simulink library "sm_pump_triplex_lib"  (R2025a)
settings: Solver=VariableStepAuto  StartTime=0.0  StopTime=10.0  RelTol=1e-3
undefined symbols (not defined in the file): cyl_stroke_P, seal_leak_vis_clr_P, seal_leak_vis_len_P, seal_leak_vis_rad_P, TRP_Par, X, Y, Z
libraries: sm_lib x30, fl_lib x10, SimscapeFluids_lib x4, nesl_utility x4
(part 1 of 2)
Description:
  | Copyright 2017-2025 The MathWorks, Inc.
settings Model: Creator=smiller  LastModifiedBy=smiller
settings SolverCC: AlgebraicLoopSolver=TrustRegion
settings DataIOCC: ReturnWorkspaceOutputs=off
settings OptimizationCC: ReuseModelBlockBuffer=off
settings DebuggingCC: UnconnectedInputMsg=warning  UnconnectedOutputMsg=warning  UnconnectedLineMsg=warning  PregeneratedLibrarySubsystemCodeDiagnostic=none  ArithmeticOperatorsInVariantConditions=warning
settings ModelReferenceCC: EnableRefExpFcnMdlSchedulingChecks=on
settings SFSimCC: SimUseLocalCustomCode=off  CustomCodeUndefinedFunction=UseInterfaceOnly
settings RTWCC: RTWUseLocalCustomCode=off  GPUComputeCapability=3.5  DLArmComputeVersion=19.05

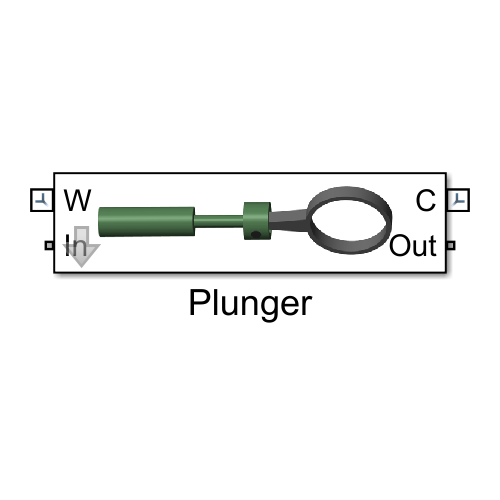
[thumbnail: Simulink's stored preview of the top-level diagram]
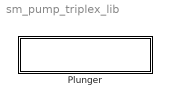
== system sm_pump_triplex_lib ==
  Plunger : Subsystem  mask(Hydraulic Plunger){cyl_gap=TRP_Par.Cylinder.gap, cyl_rad_out=TRP_Par.Cylinder.rad_outer, cyl_len=TRP_Par.Plunger.len, cyl_stroke=cyl_stroke_P, cyl_rad_in=0, cyl_xc_rev=0, cyl_frict_brkway_frc=TRP_Par.Cylinder.Friction.BrkFrc, cyl_frict_brkway_vel=TRP_Par.Cylinder.Friction.BrkVel, cyl_frict_col_frc=TRP_Par.Cylinder.Friction.ColFrc, cyl_frict_visc_coef=TRP_Par.Cylinder.Friction.ViscCo, cyl_rho=TRP_Par.Cylinder.rho, cyl_clr=TRP_Par.Cylinder.clr, cyl_opc=TRP_Par.Cylinder.opc, plgB_len=TRP_Par.Plunger.len, plgB_rad=TRP_Par.Plunger.rad, stem_len=TRP_Par.Stem.len, stem_rad=TRP_Par.Stem.rad, pin_len=TRP_Par.Pin.len, pin_rad=TRP_Par.Pin.rad, cup_rad_out=TRP_Par.StemCup.rad, cup_thk=TRP_Par.StemCup.wall, cup_len=TRP_Par.StemCup.len, cup_pinOffset=TRP_Par.StemCup.pinOffset, cup_rad_in=0, plg_rho=TRP_Par.Plunger.rho, plg_clr=TRP_Par.Plunger.clr, plg_opc=TRP_Par.Plunger.opc, conrod_len=TRP_Par.ConRod.len, conrod_web_widP=TRP_Par.ConRod.W1, conrod_web_widC=TRP_Par.ConRod.W2, conrod_web_offC=0, conrod_web_offP=0, conrod_web_len=0, conrod_web_xc=0, conrod_ringC_wid=TRP_Par.ConRod.R2.width, conrod_ringP_wid=TRP_Par.ConRod.R1.width, crank_shaft_rad=TRP_Par.Crank.Shaft.rad, conrod_ringC_or=0, conrod_ringP_or=0, conrod_ringC_xc_rev=0, conrod_ringP_xc_rev=0, conrod_thk=TRP_Par.ConRod.hei, conrod_rho=TRP_Par.ConRod.rho, conrod_clr=TRP_Par.ConRod.clr, conrod_opc=TRP_Par.ConRod.opc, chkv_in_maxA=TRP_Par.Check_Valve.In.Max_Area, chkv_out_maxA=TRP_Par.Check_Valve.Out.Max_Area, chkv_press_set_popup=Set in Mask, chkv_in_crkP=TRP_Par.Check_Valve.In.Crack_Pr, chkv_out_crkP=TRP_Par.Check_Valve.Out.Crack_Pr, chkv_in_maxOpenP=TRP_Par.Check_Valve.In.Max_Open_Pr, chkv_out_maxOpenP=TRP_Par.Check_Valve.Out.Max_Open_Pr, chkv_vis_popup=Off, chkv_vis_rad_in=0, chkv_vis_rad_out=0, chkv_vis_clr_in=0, chkv_vis_clr_out=0, leak_cyl_popup=Off, leak_cyl_area=TRP_Par.Check_Valve.In.Max_Area*0.05, block_in_popup=Off, block_in_factor=0.8, seal_leak_vis_len=seal_leak_vis_len_P, seal_leak_vis_rad=seal_leak_vis_rad_P, seal_leak_vis_clr=seal_leak_vis_clr_P, seal_leak_vis_opc=0, inlet_obstr_len=TRP_Par.Manifold.Inlet.obstr.len, inlet_obstr_rad=TRP_Par.Manifold.Inlet.rad, inlet_obstr_xc_rev=0, inlet_obstr_clr=TRP_Par.Manifold.Inlet.obstr.clr, inlet_obstr_opc=1}
      mask prompts: cyl_gap "Gap (m)"; cyl_rad_out "Outer radius (m)"; cyl_len "Length (m)"; cyl_stroke "Stroke (m)"; cyl_rad_in "Inner radius (m)"; cyl_xc_rev "Revolution Cross Section (m)"; cyl_frict_brkway_frc "Breakaway Friction Force (N)"; cyl_frict_brkway_vel "Breakaway Friction Velocity (m/s)"; cyl_frict_col_frc "Coulomb Friction Force (N)"; cyl_frict_visc_coef "Viscous Friction Coeff (N/(m/s))"; cyl_rho "Density (kg/m^3)"; cyl_clr "Color [RGB]"; cyl_opc "Opacity (0-1)"; cup_rad_out "Outer Radius (m)"; cup_thk "Wall Thickness (m)"; cup_len "Length(m)"; cup_pinOffset "Pin Offset (m)"; cup_rad_in "Inner Radius (m)"; plg_rho "Density (kg/m^3)"; plg_clr "Color [RGB]"; plg_opc "Opacity (0-1)"; conrod_len "Length, center-center (m)"; conrod_web_widP "Width, pin end (m)"; conrod_web_widC "Width, crank end (m)"; conrod_web_offC "Offset to shaft center (m)"; conrod_web_offP "Offset to pin center (m)"; conrod_web_len "Length web (m)"; conrod_web_xc "Extrusion cross section (m)"; conrod_ringC_wid "Crank Ring Width (m)"; conrod_ringP_wid "Pin Ring Width (m)"; crank_shaft_rad "Crank Shaft Radius (m)"; conrod_ringC_or "Outer Radius, Crank Ring"; conrod_ringP_or "Inner Radius, Pin Ring"; conrod_ringC_xc_rev "Crank Ring Cross Section (m)"; conrod_ringP_xc_rev "Pin Ring Cross Section (m)"; conrod_thk "Thickness (m)"; conrod_rho "Density (kg/m^3)"; conrod_clr "Color [RGB]"; conrod_opc "Opacity (0-1)"; chkv_press_set_popup "Pressure Settings"; chkv_vis_popup "Valve Visualization"; leak_cyl_popup "Seal Leak"; leak_cyl_area "Leak Area (m^2)"; block_in_popup "Blocked Inlet"; block_in_factor "Area Factor (0-1)"; seal_leak_vis_len "Length (m)"; seal_leak_vis_rad "Radius (m)"; seal_leak_vis_clr "Color [RGB]"; seal_leak_vis_opc "Opacity (0-1)"; inlet_obstr_len "Length (m)"; inlet_obstr_rad "Radius (m)"; inlet_obstr_xc_rev "Cross Section (m)"; inlet_obstr_clr "Color [RGB]"; inlet_obstr_opc "Opacity (0-1)"
      mask help: Models a single hydraulic plunger with hydraulic chamber. Two check valves control flow into and out of the hydraulic chamber. Degraded behavior can be modeled by enabling seal leakage and blocked inlet on the Faults tab. When "On, Run Time" is selected, MATLAB workspace variables set the parameters so that they can be tuned using Fast Restart.
      mask init:
      | % -- Configure submodels
      | % Fault: Seal Leak
      | if(leak_cyl_popup==1)
      |     set_param([gcb '/Seal Leak'],'OverrideUsingVariant','Off');
      |     seal_leak_vis_opc = 0;
      | elseif(leak_cyl_popup==2)
      |     set_param([gcb '/Seal Leak'],'OverrideUsingVariant','On');
      |     seal_leak_vis_opc = 1;
      | elseif(leak_cyl_popup==3)
      |     set_param([gcb '/Seal Leak'],'OverrideUsingVariant','Tune');
      |     seal_leak_vis_opc = 1;
      | end
      | 
      | % Fault: Blocked Inlet
      | inlet_obstr_xc_rev = [...
      |     inlet_obstr_rad                  -inlet_obstr_len/2;
      |     inlet_obstr_rad                   inlet_obstr_len/2;
      |     inlet_obstr_rad*block_in_factor   inlet_obstr_len/2;
      |     inlet_obstr_rad*block_in_factor  -inlet_obstr_len/2];
      | if(block_in_popup==1)
      |     set_param([gcb '/Check Valve Inlet'],...
      |         'area_max','chkv_in_maxA',...
      |         'area_max_conf','compiletime',...
      |         'BackgroundColor','[1 1 1]');
      |     inlet_obstr_opc = 0;
      | elseif(block_in_popup==2)
      |     set_param([gcb '/Check Valve Inlet'],...
      |         'area_max','chkv_in_maxA*block_in_factor',...
      |         'area_max_conf','compiletime',...
      |         'BackgroundColor','[1 0.9 0.9]');
      |     inlet_obstr_opc = 1;
      | elseif(block_in_popup==3)
      |     set_param([gcb '/Check Valve Inlet'],...
      |         'area_max','chkv_in_maxA_WKSP*block_in_factor_WKSP',...
      |         'area_max_conf','runtime',...
      |         'BackgroundColor','[1 0.9 0.9]');
      |     inlet_obstr_opc = 1;
      | end
      | 
      | % Parameter tuning: Check valve pressure settings
      | 
      | if(chkv_press_set_popup==1)
      |     set_param([gcb '/Check Valve Inlet'],...
      |         'p_crack_differential','chkv_in_crkP',...
      |         'p_crack_differential_conf','compiletime',...
      |         'press_max_differential','chkv_in_maxOpenP',...
      |         'press_max_differential_conf','compiletime');
      |     set_param([gcb '/Check Valve Outlet'],...
      |         'p_crack_differential','chkv_out_crkP',...
      |         'p_crack_differential_conf','compiletime',...
      |         'press_max_differential','chkv_out_maxOpenP',...
      |         'press_max_differential_conf','compiletime');
      | elseif(chkv_press_set_popup==2)
      |     set_param([gcb '/Check Valve Inlet'],...
      |         'p_crack_differential','chkv_all_crkP_WKSP',...
      |         'p_crack_differential_conf','runtime',...
      |         'press_max_differential','chkv_all_maxOpenP_WKSP',...
      |         'press_max_differential_conf','runtime');
      |     set_param([gcb '/Check Valve Outlet'],...
      |         'p_crack_differential','chkv_all_crkP_WKSP',...
      |         'p_crack_differential_conf','runtime',...
      |         'press_max_differential','chkv_all_maxOpenP_WKSP',...
      |         'press_max_differential_conf','runtime');
      | end
      | 
      | % Turn on/off visualization
      | if(chkv_vis_popup==1)
      |     set_param([gcb '/Valve Visual'],'OverrideUsingVariant','Off');
      | elseif(chkv_vis_popup==2)
      |     set_param([gcb '/Valve Visual'],'OverrideUsingVariant','On');
      | end
      | 
      | % -- Calculate derived parameters
      | % Cylinder: derived dimensions
      | cyl_rad_in  = plgB_rad + cyl_gap;
      | 
      | % Cylinder: cross-section for rev
      | cyl_xc_rev = [...
      |     cyl_rad_out  -cyl_len/2
      |     cyl_rad_out   cyl_len/2
      |     cyl_rad_in    cyl_len/2
      |     cyl_rad_in   -cyl_len/2];
      | 
      | % Stem Cup: cross-section for rev
      | cup_rad_in = cup_rad_out-cup_thk;
      | cup_xc_rev = [...
      |     cup_rad_out  -cup_len/2
      |     cup_rad_out   cup_len/2
      |     cup_rad_in    cup_len/2
      |     cup_rad_in   -cup_len/2];
      | 
      | % Connecting Rod, Crank Ring: cross-section for rev
      | conrod_ringC_or = crank_shaft_rad + conrod_ringC_wid;
      | conrod_ringC_xc_rev = [...
      |     conrod_ringC_or -conrod_thk/2*1.005;
      |     conrod_ringC_or  conrod_thk/2*1.005;
      |     crank_shaft_rad  conrod_thk/2*1.005;
      |     crank_shaft_rad -conrod_thk/2*1.005];
      | 
      | % Connecting Rod, Pin ring: cross-section for rev
      | conrod_ringP_or = pin_rad + conrod_ringP_wid;
      | conrod_ringP_xc_rev = [...
      |     conrod_ringP_or -conrod_thk/2*1.005;
      |     conrod_ringP_or  conrod_thk/2*1.005;
      |     pin_rad          conrod_thk/2*1.005;
      |     pin_rad         -conrod_thk/2*1.005];
      | 
      | % Connecting Rod, Web: cross-section for extrusion
      | conrod_web_offC = crank_shaft_rad + conrod_ringC_wid/2;
      | conrod_web_offP = pin_rad         + conrod_ringP_wid/2;
      | conrod_web_len  = conrod_len - conrod_web_offP - conrod_web_offC;
      | conrod_web_xc = [...
      |     -conrod_web_len -conrod_web_widC;
      |     conrod_web_len -conrod_web_widP;
      |     conrod_web_len  conrod_web_widP;
      |     -conrod_web_len  conrod_web_widC]/2;
      mask TypeOptions chkv_press_set_popup: Set in Mask | Tune at Run Time
      mask Callback chkv_press_set_popup:
      | maskObj = Simulink.Mask.get(gcb);
      | 
      | crPrP_h = maskObj.getDialogControl('text_open_crkP');
      | crMxP_h = maskObj.getDialogControl('text_open_maxOpenP');
      | crPIn_h = maskObj.getParameter('chkv_in_crkP');
      | crPOu_h = maskObj.getParameter('chkv_out_crkP');
      | mxPIn_h = maskObj.getParameter('chkv_in_maxOpenP');
      | mxPOu_h = maskObj.getParameter('chkv_out_maxOpenP');
      | 
      | allTxt_h = maskObj.getDialogControl('chkv_pres_set_all_tune_text');
      | 
      | temp_PressSetTune = get_param(gcb,'chkv_press_set_popup');
      | 
      | if (strcmp(temp_PressSetTune,'Set in Mask'))
      |     crPrP_h.Visible = 'on';
      |     crMxP_h.Visible = 'on';
      |     crPIn_h.Visible = 'on';
      |     crPOu_h.Visible = 'on';
      |     mxPIn_h.Visible = 'on';
      |     mxPOu_h.Visible = 'on';
      |     allTxt_h.Visible = 'off';
      |     outTxt_h.Visible = 'off';
      | else
      |     crPrP_h.Visible = 'off';
      |     crMxP_h.Visible = 'off';
      |     crPIn_h.Visible = 'off';
      |     crPOu_h.Visible = 'off';
      |     mxPIn_h.Visible = 'off';
      |     mxPOu_h.Visible = 'off';
      |     allTxt_h.Visible = 'on';
      |     outTxt_h.Visible = 'on';
      | end
      | clear maskObj temp_PressSetTune
      | clear crPrP_h crMxP_h crPIn_h crPOu_h mxPIn_h mxPOu_h
      | clear allTxt_h
      mask TypeOptions chkv_vis_popup: Off | On
      mask TypeOptions leak_cyl_popup: Off | On | On, Run Time
      mask Callback leak_cyl_popup:
      | maskObj = Simulink.Mask.get(gcb);
      | leak_area_h = maskObj.getParameter('leak_cyl_area');
      | leak_text_h = maskObj.getDialogControl('leak_cyl_tune_text');
      | if (strcmp(get_param(gcb,'leak_cyl_popup'),'Off'))
      |     leak_area_h.Visible = 'off';
      |     leak_text_h.Visible = 'off';
      | elseif (strcmp(get_param(gcb,'leak_cyl_popup'),'On'))
      |     leak_area_h.Visible = 'on';
      |     leak_text_h.Visible = 'off';
      | elseif (strcmp(get_param(gcb,'leak_cyl_popup'),'On, Run Time'))
      |     leak_area_h.Visible = 'off';
      |     leak_text_h.Visible = 'on';
      | end
      | %clear maskObj leak_area_h leak_text_h
      mask TypeOptions block_in_popup: Off | On | On, Run Time
      mask Callback block_in_popup:
      | maskObj = Simulink.Mask.get(gcb);
      | block_fctr_h = maskObj.getParameter('block_in_factor');
      | block_text_h = maskObj.getDialogControl('block_in_tune_text');
      | if (strcmp(get_param(gcb,'block_in_popup'),'Off'))
      |     block_fctr_h.Visible = 'off';
      |     block_text_h.Visible = 'off';
      | elseif (strcmp(get_param(gcb,'block_in_popup'),'On'))
      |     block_fctr_h.Visible = 'on';
      |     block_text_h.Visible = 'off';
      | elseif (strcmp(get_param(gcb,'block_in_popup'),'On, Run Time'))
      |     block_fctr_h.Visible = 'off';
      |     block_text_h.Visible = 'on';
      | end
      | clear maskObj block_fctr_h block_text_h
      mask DialogControl tab_cylinder Prompt: Cylinder
      mask DialogControl cont_dims Prompt: Dimensions
      mask DialogControl cont_friction Prompt: Friction
      mask DialogControl cont_cyl_vis Prompt: Cylinder Visualization
      mask DialogControl tab_plunger Prompt: Plunger
      mask DialogControl text_length Prompt: Length (m)
      mask DialogControl text_radius Prompt: Radius (m)
      mask DialogControl text_base Prompt: Base
      mask DialogControl text_stem Prompt: Stem
      mask DialogControl text_pin Prompt: Pin
      mask DialogControl cont_cup Prompt: Cup
      mask DialogControl cont_plg_vis Prompt: Plunger Visualization
      mask DialogControl tab_conrod Prompt: Rod
      mask DialogControl cont_conrodWeb Prompt: Web
      mask DialogControl cont_conrodRings Prompt: Rings
      mask DialogControl cont_conrod_vis Prompt: Rod Visualization
      mask DialogControl tab_valves Prompt: Valves
      mask DialogControl text_open_inlet Prompt: Inlet
      mask DialogControl text_open_outlet Prompt: Outlet
      mask DialogControl text_open_maxA Prompt: Max Area (m)
      mask DialogControl text_open_crkP Prompt: Crack. Pr (Pa)
      mask DialogControl text_open_maxOpenP Prompt: Max Pr. (Pa)
      mask DialogControl chkv_pres_set_all_tune_text Prompt: Set >> chkv_all_crkP_WKSP, chkv_all_maxOpenP_WKSP
      mask DialogControl cont_valve_vis Prompt: Visualization Settings
      mask DialogControl text_valvis_inlet Prompt: Inlet
      mask DialogControl text_valvis_out Prompt: Outlet
      mask DialogControl text_valvis_rad Prompt: Radius (m)
      mask DialogControl text_valvis_clr Prompt: Color [RGB]
      mask DialogControl tab_faults Prompt: Faults
      mask DialogControl leak_cyl_tune_text Prompt: Set >> leak_cyl_area_WKSP
      mask DialogControl block_in_tune_text Prompt: Set >> block_in_factor_WKSP, chkv_out_maxA_WKSP
      mask DialogControl cont_seal_leak_vis Prompt: Seal Leak Visualization
      mask DialogControl cont_blocked_line_vis Prompt: Blocked Line Visualization
      mask Display: image('sm_pump_triplex_Plunger_IMAGE.png');

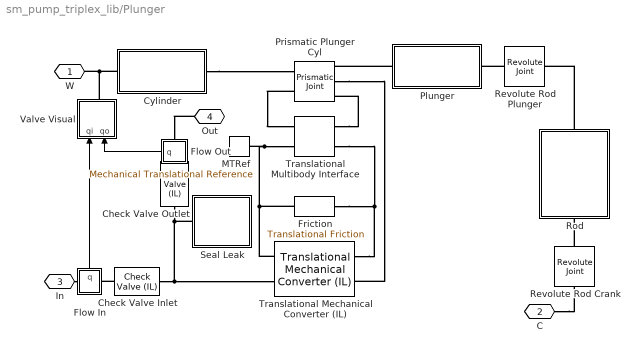
== system sm_pump_triplex_lib/Plunger ==
  Check Valve Outlet : SimscapeFluids_lib/Isothermal Liquid/Valves & Orifices/Directional Control Valves/Check Valve (IL)  opening_spec=fluids.isothermal_liquid.valves_orifices.enum.PressureOpeningSpec.Linear  pressure_control_spec=fluids.isothermal_liquid.valves_orifices.enum.pressure_control_spec.dp  p_crack_differential=chkv_out_crkP Pa  p_crack_gauge=0.1 MPa  press_max_differential=chkv_out_maxOpenP Pa  press_max_gauge=0.2 MPa  area_max=chkv_out_maxA m^2  area_leak=1e-12 m^2  p_diff_TLU=[0.01 : 0.01 : 0.1] MPa  valve_area_TLU=[1e-10, 1e-05, 2e-05, 3e-05, 4e-05, 5e-05, 6e-05, 7.5e-05, 8.5e-05, .0001] m^2  vol_flow_TLU=[.000358, .045, .11, .191, .284, .39, .505, .63, .764, .905] .* 1e-3 m^3/s  area=inf m^2  Cd=0.7  Re_c=150  smoothing_factor=0  pressure_recovery=false  opening_dynamics=0  tau=0.1 s
      settings: LibrarySourceBlock=sh_lib/Valves/Directional Valves/Check Valve  InternalSimscapePortConfiguration="{\"Bottom\":[],\"Left\":[{\"id\":\"A\",\"label\":\"A\",\"type\":\"foundation.isothermal_liquid.isothermal_liquid\"}],\"Right\":[{\"id\":\"B\",\"label\":\"B\",\"type\":\"foundation.isothermal_liquid.isothermal_liquid\"}],\"Top\":[]}"
  Check Valve Inlet : SimscapeFluids_lib/Isothermal Liquid/Valves & Orifices/Directional Control Valves/Check Valve (IL)  opening_spec=fluids.isothermal_liquid.valves_orifices.enum.PressureOpeningSpec.Linear  pressure_control_spec=fluids.isothermal_liquid.valves_orifices.enum.pressure_control_spec.dp  p_crack_differential=chkv_in_crkP Pa  p_crack_gauge=0.1 MPa  press_max_differential=chkv_in_maxOpenP Pa  press_max_gauge=0.2 MPa  area_max=chkv_in_maxA m^2  area_leak=1e-12 m^2  p_diff_TLU=[0.01 : 0.01 : 0.1] MPa  valve_area_TLU=[1e-10, 1e-05, 2e-05, 3e-05, 4e-05, 5e-05, 6e-05, 7.5e-05, 8.5e-05, .0001] m^2  vol_flow_TLU=[.000358, .045, .11, .191, .284, .39, .505, .63, .764, .905] .* 1e-3 m^3/s  area=inf m^2  Cd=0.7  Re_c=150  smoothing_factor=0  pressure_recovery=false  opening_dynamics=0  tau=0.1 s
      settings: LibrarySourceBlock=sh_lib/Valves/Directional Valves/Check Valve  InternalSimscapePortConfiguration="{\"Bottom\":[],\"Left\":[{\"id\":\"A\",\"label\":\"A\",\"type\":\"foundation.isothermal_liquid.isothermal_liquid\"}],\"Right\":[{\"id\":\"B\",\"label\":\"B\",\"type\":\"foundation.isothermal_liquid.isothermal_liquid\"}],\"Top\":[]}"
  Cylinder : Subsystem
      mask Display: image('sm_pump_triplex_Cylinder_IMAGE.png');
  Flow In : Subsystem
      settings: PortSchema="{\"entries\":[{\"content\":{\"sides\":[{\"content\":{\"connectorIds\":[\"LConn1\"]},\"type\":\"ConnectorPlacement.EquallySpacedRectSide\",\"uuid\":\"d8890d1f-efe5-450c-a9d1-631aa55099a3\"},{\"content\":{\"connectorIds\":[\"RConn1\"],\"side\":\"RIGHT\"},\"type\":\"ConnectorPlacement.EquallySpacedRectSide\",\"uuid\":\"e7902446-afb0-4dff-a73a-74a0f518c034\"},{\"content\":{\"connectorIds\":[\"Out1\"],\"side\":\"TOP\"},\"type\":\"ConnectorPlacement.EquallySpacedRectSide\",\"uuid\":\"0f4acc62-ad4e-4cfb-b3e1-af6631ecf4f2\"}]},\"type\":\"ConnectorPlacement.EquallySpacedConnector\",\"uuid\":\"0d068d5e-401c-4540-957a-9d86136fa137\"}],\"packageUris\":[\"http://schema.mathworks.com/mf0/Connector/R2020b\"],\"version\":\"1.0\"}"
      mask Display: image('sm_pump_triplex_FlowSensor_IMAGE.png');
  Flow Out : Subsystem
      settings: PortSchema="{\"entries\":[{\"content\":{\"sides\":[{\"content\":{\"connectorIds\":[\"LConn1\"]},\"type\":\"ConnectorPlacement.EquallySpacedRectSide\",\"uuid\":\"331f03af-e47d-4d6f-a6dc-b815d7a097d8\"},{\"content\":{\"connectorIds\":[\"RConn1\"],\"side\":\"RIGHT\"},\"type\":\"ConnectorPlacement.EquallySpacedRectSide\",\"uuid\":\"dacb2701-8592-47cf-bd72-a70e874db693\"},{\"content\":{\"connectorIds\":[\"Out1\"],\"side\":\"TOP\"},\"type\":\"ConnectorPlacement.EquallySpacedRectSide\",\"uuid\":\"5cbd76fa-51da-45d8-8d23-e2a6e5c372b8\"}]},\"type\":\"ConnectorPlacement.EquallySpacedConnector\",\"uuid\":\"f481fdea-1e41-400e-8027-eeb12cc1f64b\"}],\"packageUris\":[\"http://schema.mathworks.com/mf0/Connector/R2020b\"],\"version\":\"1.0\"}"
      mask Display: image('sm_pump_triplex_FlowSensor_L_IMAGE.png');
  Friction : fl_lib/Mechanical/Translational Elements/Translational Friction  brkwy_frc=cyl_frict_brkway_frc N  brkwy_vel=cyl_frict_brkway_vel m/s  Col_frc=cyl_frict_col_frc N  visc_coef=cyl_frict_visc_coef N/(m/s)  v_specify=off  v_priority=None  v=0 m/s  v_nominal_specify=off  v_nominal_value=1  v_nominal_unit=m/s  f_specify=off  f_priority=None  f=0 N  f_nominal_specify=off  f_nominal_value=1  f_nominal_unit=N
      settings: InternalSimscapePortConfiguration="{\"Bottom\":[],\"Left\":[{\"id\":\"R\",\"label\":\"R\",\"type\":\"foundation.mechanical.translational.translational\"}],\"Right\":[{\"id\":\"C\",\"label\":\"C\",\"type\":\"foundation.mechanical.translational.translational\"}],\"Top\":[]}"
  MTRef : fl_lib/Mechanical/Translational Elements/Mechanical Translational Reference
  Plunger : Subsystem
      mask Display: image('sm_pump_triplex_PlungerPart_IMAGE.png');
  Prismatic Plunger Cyl : sm_lib/Joints/Prismatic Joint  JointMode=Normal  CompositeWrenchDir=FollowerOnBase  CompositeWrenchFrame=BaseFrame  SenseConstraintForce=off  SenseConstraintTorque=off  SenseTotalForce=off  SenseTotalTorque=off  PositionTargetSpecify=off  PositionTargetPriority=High  PositionTargetValue=0  PositionTargetValueUnits=m  VelocityTargetSpecify=off  VelocityTargetPriority=High  VelocityTargetValue=0  VelocityTargetValueUnits=m/s  EquilibriumPosition=0  EquilibriumPositionUnits=m  SpringStiffness=0  SpringStiffnessUnits=N/m  DampingCoefficient=0  DampingCoefficientUnits=N/(m/s)  LowerLimitSpecify=off  LowerLimitBound=-1  LowerLimitBoundUnits=m  LowerLimitStiffness=1e6  LowerLimitStiffnessUnits=N/m  LowerLimitDamping=1e3  LowerLimitDampingUnits=N/(m/s)  LowerLimitTransitionRegionWidth=1e-4  LowerLimitTransitionRegionWidthUnits=m  UpperLimitSpecify=off  UpperLimitBound=1  UpperLimitBoundUnits=m  UpperLimitStiffness=1e6  UpperLimitStiffnessUnits=N/m  UpperLimitDamping=1e3  UpperLimitDampingUnits=N/(m/s)  UpperLimitTransitionRegionWidth=1e-4  UpperLimitTransitionRegionWidthUnits=m  TorqueActuationMode=InputTorque  MotionActuationMode=ComputedMotion  SensePosition=on  SenseVelocity=on  SenseAcceleration=off  SenseTorqueForce=off  SenseLowerLimitTorqueForce=off  SenseUpperLimitTorqueForce=off
  Revolute Rod Crank : sm_lib/Joints/Revolute Joint  JointMode=Normal  CompositeWrenchDir=FollowerOnBase  CompositeWrenchFrame=BaseFrame  SenseConstraintForce=off  SenseConstraintTorque=off  SenseTotalForce=off  SenseTotalTorque=off  PositionTargetSpecify=off  PositionTargetPriority=High  PositionTargetValue=0  PositionTargetValueUnits=deg  VelocityTargetSpecify=off  VelocityTargetPriority=High  VelocityTargetValue=0  VelocityTargetValueUnits=deg/s  EquilibriumPosition=0  EquilibriumPositionUnits=deg  SpringStiffness=0  SpringStiffnessUnits=N*m/deg  DampingCoefficient=0  DampingCoefficientUnits=N*m/(deg/s)  LowerLimitSpecify=off  LowerLimitBound=-90  LowerLimitBoundUnits=deg  LowerLimitStiffness=1e4  LowerLimitStiffnessUnits=N*m/deg  LowerLimitDamping=10  LowerLimitDampingUnits=N*m/(deg/s)  LowerLimitTransitionRegionWidth=0.1  LowerLimitTransitionRegionWidthUnits=deg  UpperLimitSpecify=off  UpperLimitBound=90  UpperLimitBoundUnits=deg  UpperLimitStiffness=1e4  UpperLimitStiffnessUnits=N*m/deg  UpperLimitDamping=10  UpperLimitDampingUnits=N*m/(deg/s)  UpperLimitTransitionRegionWidth=0.1  UpperLimitTransitionRegionWidthUnits=deg  TorqueActuationMode=NoTorque  MotionActuationMode=ComputedMotion  SensePosition=off  SenseVelocity=off  SenseAcceleration=off  SenseTorqueForce=off  SenseLowerLimitTorqueForce=off  SenseUpperLimitTorqueForce=off
  Revolute Rod Plunger : sm_lib/Joints/Revolute Joint  JointMode=Normal  CompositeWrenchDir=FollowerOnBase  CompositeWrenchFrame=BaseFrame  SenseConstraintForce=off  SenseConstraintTorque=off  SenseTotalForce=off  SenseTotalTorque=off  PositionTargetSpecify=off  PositionTargetPriority=High  PositionTargetValue=0  PositionTargetValueUnits=deg  VelocityTargetSpecify=off  VelocityTargetPriority=High  VelocityTargetValue=0  VelocityTargetValueUnits=deg/s  EquilibriumPosition=0  EquilibriumPositionUnits=deg  SpringStiffness=0  SpringStiffnessUnits=N*m/deg  DampingCoefficient=0  DampingCoefficientUnits=N*m/(deg/s)  LowerLimitSpecify=off  LowerLimitBound=-90  LowerLimitBoundUnits=deg  LowerLimitStiffness=1e4  LowerLimitStiffnessUnits=N*m/deg  LowerLimitDamping=10  LowerLimitDampingUnits=N*m/(deg/s)  LowerLimitTransitionRegionWidth=0.1  LowerLimitTransitionRegionWidthUnits=deg  UpperLimitSpecify=off  UpperLimitBound=90  UpperLimitBoundUnits=deg  UpperLimitStiffness=1e4  UpperLimitStiffnessUnits=N*m/deg  UpperLimitDamping=10  UpperLimitDampingUnits=N*m/(deg/s)  UpperLimitTransitionRegionWidth=0.1  UpperLimitTransitionRegionWidthUnits=deg  TorqueActuationMode=NoTorque  MotionActuationMode=ComputedMotion  SensePosition=off  SenseVelocity=off  SenseAcceleration=off  SenseTorqueForce=off  SenseLowerLimitTorqueForce=off  SenseUpperLimitTorqueForce=off
  Rod : Subsystem
      mask Display: image('sm_pump_triplex_Rod_IMAGE.png');
  Seal Leak : Subsystem  Variant=on  VariantControlMode=label  VariantControl=Variant1  LabelModeActiveChoice=Off
      settings: AttributesFormatString=%<ActiveVariant>
      mask Display:
      | blk = sm_pump_triplex_activeVariantBlock(gcb);
      | eval(get_param(blk, 'MaskDisplay'));
  Translational Mechanical Converter (IL) : fl_lib/Isothermal Liquid/Elements/Translational Mechanical Converter (IL)  mech_orientation=foundation.enum.MechOrientationTranslational.Positive  displacement_spec=foundation.enum.DisplacementSpec.InputSignal  x0=0 m  interface_area=pi*plgB_rad^2 m^2  dead_volume=8.0000e-06 m^3  pressure_spec=foundation.enum.pressure_spec.atmospheric  environment_pressure=0.101325 MPa  dynamic_compressibility=simscape.enum.onoff.on  p0=0.101325 MPa  p_nominal=0.101325 MPa
      settings: InternalSimscapePortConfiguration="{\"Bottom\":[],\"Left\":[{\"id\":\"A\",\"label\":\"A\",\"type\":\"foundation.isothermal_liquid.isothermal_liquid\"},{\"id\":\"C\",\"label\":\"C\",\"type\":\"foundation.mechanical.translational.translational\"}],\"Right\":[{\"id\":\"p_in\",\"label\":\"p\",\"type\":\"input\"},{\"id\":\"R\",\"label\":\"R\",\"type\":\"foundation.mechanical.translational.translational\"}],\"Top\":[]}"
  Translational Multibody Interface : fl_lib/Mechanical/Multibody Interfaces/Translational Multibody Interface
  Valve Visual : Subsystem  Variant=on  VariantControlMode=label  VariantControl=Variant1  LabelModeActiveChoice=Off
      settings: AttributesFormatString=%<ActiveVariant>
      mask Display:
      | blk = sm_pump_triplex_activeVariantBlock(gcb);
      | eval(get_param(blk, 'MaskDisplay'));
  W : PMIOPort  Side=Left
  C : PMIOPort  Port=2  Side=Right
  In : PMIOPort  Port=3  Side=Left
  Out : PMIOPort  Port=4  Side=Right
  wires:
  Flow In/1(q) -> Valve Visual/1("qi ")
  Flow Out/1(q) -> Valve Visual/2("qo ")
  connections:
  Prismatic Plunger Cyl/LConn2 -- Translational Multibody Interface/LConn1
  Translational Multibody Interface/RConn1 -- Prismatic Plunger Cyl/RConn3
  Prismatic Plunger Cyl/RConn2 -- Translational Mechanical Converter (IL)/RConn1
  Revolute Rod Plunger/LConn1 -- Plunger/RConn1
  C/RConn1 -- Revolute Rod Crank/RConn1
  Revolute Rod Crank/LConn1 -- Rod/RConn1
  Plunger/LConn1 -- Prismatic Plunger Cyl/RConn1
  Rod/LConn1 -- Revolute Rod Plunger/RConn1
  Cylinder/RConn1 -- Prismatic Plunger Cyl/LConn1
  Check Valve Inlet/RConn1 -- Translational Mechanical Converter (IL)/LConn1 -- Seal Leak/LConn1 -- Check Valve Outlet/LConn1
  In/RConn1 -- Flow In/RConn1
  Check Valve Inlet/LConn1 -- Flow In/LConn1
  Out/RConn1 -- Flow Out/RConn1
  W/RConn1 -- Cylinder/LConn1 -- Valve Visual/RConn1
  Flow Out/LConn1 -- Check Valve Outlet/RConn1
  Friction/RConn1 -- MTRef/LConn1 -- Translational Multibody Interface/LConn2 -- Translational Mechanical Converter (IL)/LConn2
  Friction/LConn1 -- Translational Mechanical Converter (IL)/RConn2 -- Translational Multibody Interface/RConn2

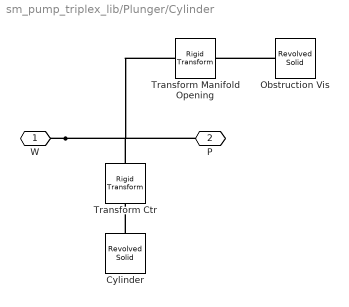
== system sm_pump_triplex_lib/Plunger/Cylinder ==
  Cylinder : sm_lib/Body Elements/Revolved Solid  RevolutionCrossSection=cyl_xc_rev  RevolutionCrossSectionUnits=m  RevolutionExtent=Full  RevolutionAngle=180  RevolutionAngleUnits=deg  ExportConvexHullGeometry=off  InertiaType=CalculateFromGeometry  BasedOnType=Density  Density=cyl_rho  DensityUnits=kg/m^3  Mass=1  MassUnits=kg  CenterOfMass=[0 0 0]  CenterOfMassUnits=m  MomentsOfInertia=[1 1 1]  MomentsOfInertiaUnits=kg*m^2  ProductsOfInertia=[1 1 1]  ProductsOfInertiaUnits=kg*m^2  GraphicType=FromGeometry  MarkerShape=Sphere  MarkerSize=10  GraphicVisPropType=SimpleVisualProperties  GraphicDiffuseColor=cyl_clr  GraphicOpacity=cyl_opc  GraphicSpecularColor=[0.5 0.5 0.5 1.0]  GraphicAmbientColor=[0.15 0.15 0.15 1.0]  GraphicEmissiveColor=[0.0 0.0 0.0 1.0]  GraphicShininess=75  DoExposeReferenceFrame=on  SerializedFrames=<Frames/>
  Obstruction Vis : sm_lib/Body Elements/Revolved Solid  RevolutionCrossSection=inlet_obstr_xc_rev  RevolutionCrossSectionUnits=m  RevolutionExtent=Full  RevolutionAngle=180  RevolutionAngleUnits=deg  ExportConvexHullGeometry=off  InertiaType=CalculateFromGeometry  BasedOnType=Density  Density=0.001  DensityUnits=kg/m^3  Mass=1  MassUnits=kg  CenterOfMass=[0 0 0]  CenterOfMassUnits=m  MomentsOfInertia=[1 1 1]  MomentsOfInertiaUnits=kg*m^2  ProductsOfInertia=[1 1 1]  ProductsOfInertiaUnits=kg*m^2  GraphicType=FromGeometry  MarkerShape=Sphere  MarkerSize=10  GraphicVisPropType=SimpleVisualProperties  GraphicDiffuseColor=inlet_obstr_clr  GraphicOpacity=inlet_obstr_opc  GraphicSpecularColor=[0.5 0.5 0.5 1.0]  GraphicAmbientColor=[0.15 0.15 0.15 1.0]  GraphicEmissiveColor=[0.0 0.0 0.0 1.0]  GraphicShininess=75  DoExposeReferenceFrame=on  SerializedFrames=<Frames/>
  Transform Ctr : sm_lib/Frames and Transforms/Rigid Transform  RotationMethod=None  FollAlignAxisA=+X  BaseAlignAxisA=+Y  FollAlignAxisB=+Y  BaseAlignAxisB=+Z  RotationStandardAxis=+Z  RotationAngle=0.0  RotationAngleUnits=deg  RotationArbitraryAxis=[0 0 1]  RotationSequenceAxes=FollowerAxes  RotationSequence=XYX  RotationSequenceAngles=[0 0 0]  RotationSequenceAnglesUnits=deg  RotationMatrix=[1 0 0; 0 1 0; 0 0 1]  Quaternion=[1 0 0 0]  TranslationMethod=StandardAxis  TranslationCartesianOffset=[0 0 0]  TranslationCartesianOffsetUnits=m  TranslationStandardAxis=+Z  TranslationStandardOffset=cyl_len/2  TranslationStandardOffsetUnits=m  TranslationROffset=0  TranslationROffsetUnits=m  TranslationThetaOffset=0  TranslationThetaOffsetUnits=deg  TranslationZOffset=0  TranslationZOffsetUnits=m
  Transform Manifold Opening : sm_lib/Frames and Transforms/Rigid Transform  RotationMethod=None  FollAlignAxisA=+X  BaseAlignAxisA=+Y  FollAlignAxisB=+Y  BaseAlignAxisB=+Z  RotationStandardAxis=+Z  RotationAngle=0.0  RotationAngleUnits=deg  RotationArbitraryAxis=[0 0 1]  RotationSequenceAxes=FollowerAxes  RotationSequence=XYX  RotationSequenceAngles=[0 0 0]  RotationSequenceAnglesUnits=deg  RotationMatrix=[1 0 0; 0 1 0; 0 0 1]  Quaternion=[1 0 0 0]  TranslationMethod=Cartesian  TranslationCartesianOffset=[0 -0.04 -0.045-0.005]  TranslationCartesianOffsetUnits=m  TranslationStandardAxis=+Z  TranslationStandardOffset=0  TranslationStandardOffsetUnits=m  TranslationROffset=0  TranslationROffsetUnits=m  TranslationThetaOffset=0  TranslationThetaOffsetUnits=deg  TranslationZOffset=0  TranslationZOffsetUnits=m
  W : PMIOPort  Side=Left
  P : PMIOPort  Port=2  Side=Right
  connections:
  W/RConn1 -- Transform Manifold Opening/LConn1 -- P/RConn1 -- Transform Ctr/LConn1
  Cylinder/RConn1 -- Transform Ctr/RConn1
  Obstruction Vis/RConn1 -- Transform Manifold Opening/RConn1

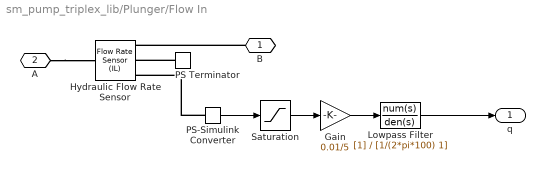
== system sm_pump_triplex_lib/Plunger/Flow In ==
  Gain : Gain  Gain=0.01/5
  Hydraulic Flow Rate Sensor : fl_lib/Isothermal Liquid/Sensors/Flow Rate Sensor (IL)  sensor_type=3
      settings: InternalSimscapePortConfiguration="{\"Bottom\":[],\"Left\":[{\"id\":\"A\",\"label\":\"A\",\"type\":\"foundation.isothermal_liquid.isothermal_liquid\"}],\"Right\":[{\"id\":\"B\",\"label\":\"B\",\"type\":\"foundation.isothermal_liquid.isothermal_liquid\"},{\"id\":\"M\",\"label\":\"M\",\"type\":\"output\"},{\"id\":\"V\",\"label\":\"V\",\"type\":\"output\"}],\"Top\":[]}"
      settings: LibrarySourceBlock=|
      | fl_lib/Hydraulic/Hydraulic Sensors/Hydraulic Flow Rate
      | Sensor
  Lowpass Filter : TransferFcn  Denominator=[1/(2*pi*100) 1]
  PS Terminator : fl_lib/Physical Signals/Sinks/PS Terminator
  PS-Simulink Converter : nesl_utility/PS-Simulink Converter  PhysicalDomain=network_engine_domain  SubClassName=ps_output  LeftPortType=input  RightPortType=output  PseudoPeriodic=off  Frequencies=[]  VectorFormat=1-D array  Unit=lpm  AffineConversion=off
  Saturation : Saturate  UpperLimit=5  LowerLimit=0  ZeroCross=off
  B : PMIOPort  Side=Left
  A : PMIOPort  Port=2  Side=Right
  q : Outport  VectorParamsAs1DForOutWhenUnconnected=off
  wires:
  PS-Simulink Converter/1 -> Saturation/1
  Saturation/1 -> Gain/1
  Gain/1 -> Lowpass Filter/1
  Lowpass Filter/1 -> q/1
  connections:
  PS-Simulink Converter/LConn1 -- Hydraulic Flow Rate Sensor/RConn3
  A/RConn1 -- Hydraulic Flow Rate Sensor/LConn1
  B/RConn1 -- Hydraulic Flow Rate Sensor/RConn1
  PS Terminator/LConn1 -- Hydraulic Flow Rate Sensor/RConn2

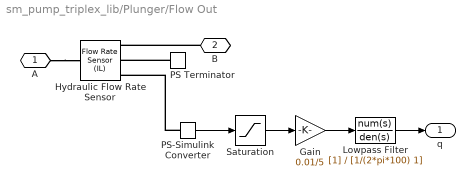
== system sm_pump_triplex_lib/Plunger/Flow Out ==
  Gain : Gain  Gain=0.01/5
  Hydraulic Flow Rate Sensor : fl_lib/Isothermal Liquid/Sensors/Flow Rate Sensor (IL)  sensor_type=3
      settings: InternalSimscapePortConfiguration="{\"Bottom\":[],\"Left\":[{\"id\":\"A\",\"label\":\"A\",\"type\":\"foundation.isothermal_liquid.isothermal_liquid\"}],\"Right\":[{\"id\":\"B\",\"label\":\"B\",\"type\":\"foundation.isothermal_liquid.isothermal_liquid\"},{\"id\":\"M\",\"label\":\"M\",\"type\":\"output\"},{\"id\":\"V\",\"label\":\"V\",\"type\":\"output\"}],\"Top\":[]}"
      settings: LibrarySourceBlock=|
      | fl_lib/Hydraulic/Hydraulic Sensors/Hydraulic Flow Rate
      | Sensor
  Lowpass Filter : TransferFcn  Denominator=[1/(2*pi*100) 1]
  PS Terminator : fl_lib/Physical Signals/Sinks/PS Terminator
  PS-Simulink Converter : nesl_utility/PS-Simulink Converter  PhysicalDomain=network_engine_domain  SubClassName=ps_output  LeftPortType=input  RightPortType=output  PseudoPeriodic=off  Frequencies=[]  VectorFormat=1-D array  Unit=lpm  AffineConversion=off
  Saturation : Saturate  UpperLimit=5  LowerLimit=0  ZeroCross=off
  A : PMIOPort  Side=Left
  B : PMIOPort  Port=2  Side=Right
  q : Outport  VectorParamsAs1DForOutWhenUnconnected=off
  wires:
  Lowpass Filter/1 -> q/1
  Gain/1 -> Lowpass Filter/1
  Saturation/1 -> Gain/1
  PS-Simulink Converter/1 -> Saturation/1
  connections:
  PS-Simulink Converter/LConn1 -- Hydraulic Flow Rate Sensor/RConn3
  A/RConn1 -- Hydraulic Flow Rate Sensor/LConn1
  B/RConn1 -- Hydraulic Flow Rate Sensor/RConn1
  PS Terminator/LConn1 -- Hydraulic Flow Rate Sensor/RConn2

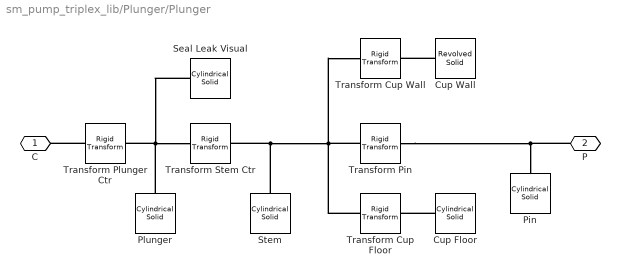
== system sm_pump_triplex_lib/Plunger/Plunger ==
  Cup Floor : sm_lib/Body Elements/Cylindrical Solid  CylinderRadius=cup_rad_out-cup_thk  CylinderRadiusUnits=m  CylinderLength=cup_thk  CylinderLengthUnits=m  ExportEntireGeometry=off  InertiaType=CalculateFromGeometry  BasedOnType=Density  Density=plg_rho  DensityUnits=kg/m^3  Mass=1  MassUnits=kg  CenterOfMass=[0 0 0]  CenterOfMassUnits=m  MomentsOfInertia=[1 1 1]  MomentsOfInertiaUnits=kg*m^2  ProductsOfInertia=[1 1 1]  ProductsOfInertiaUnits=kg*m^2  GraphicType=FromGeometry  MarkerShape=Sphere  MarkerSize=10  GraphicVisPropType=SimpleVisualProperties  GraphicDiffuseColor=plg_clr  GraphicOpacity=plg_opc  GraphicSpecularColor=[0.5 0.5 0.5 1.0]  GraphicAmbientColor=[0.15 0.15 0.15 1.0]  GraphicEmissiveColor=[0.0 0.0 0.0 1.0]  GraphicShininess=75  DoExposeReferenceFrame=on  SerializedFrames=<Frames/>
  Cup Wall : sm_lib/Body Elements/Revolved Solid  RevolutionCrossSection=cup_xc_rev  RevolutionCrossSectionUnits=m  RevolutionExtent=Full  RevolutionAngle=180  RevolutionAngleUnits=deg  ExportConvexHullGeometry=off  InertiaType=CalculateFromGeometry  BasedOnType=Density  Density=plg_rho  DensityUnits=kg/m^3  Mass=1  MassUnits=kg  CenterOfMass=[0 0 0]  CenterOfMassUnits=m  MomentsOfInertia=[1 1 1]  MomentsOfInertiaUnits=kg*m^2  ProductsOfInertia=[1 1 1]  ProductsOfInertiaUnits=kg*m^2  GraphicType=FromGeometry  MarkerShape=Sphere  MarkerSize=10  GraphicVisPropType=SimpleVisualProperties  GraphicDiffuseColor=plg_clr  GraphicOpacity=plg_opc  GraphicSpecularColor=[0.5 0.5 0.5 1.0]  GraphicAmbientColor=[0.15 0.15 0.15 1.0]  GraphicEmissiveColor=[0.0 0.0 0.0 1.0]  GraphicShininess=75  DoExposeReferenceFrame=on  SerializedFrames=<Frames/>
  Pin : sm_lib/Body Elements/Cylindrical Solid  CylinderRadius=pin_rad  CylinderRadiusUnits=m  CylinderLength=pin_len  CylinderLengthUnits=m  ExportEntireGeometry=off  InertiaType=CalculateFromGeometry  BasedOnType=Density  Density=plg_rho  DensityUnits=kg/m^3  Mass=1  MassUnits=kg  CenterOfMass=[0 0 0]  CenterOfMassUnits=m  MomentsOfInertia=[1 1 1]  MomentsOfInertiaUnits=kg*m^2  ProductsOfInertia=[1 1 1]  ProductsOfInertiaUnits=kg*m^2  GraphicType=FromGeometry  MarkerShape=Sphere  MarkerSize=10  GraphicVisPropType=SimpleVisualProperties  GraphicDiffuseColor=conrod_clr*0.5  GraphicOpacity=conrod_opc  GraphicSpecularColor=[0.5 0.5 0.5 1.0]  GraphicAmbientColor=[0.15 0.15 0.15 1.0]  GraphicEmissiveColor=[0.0 0.0 0.0 1.0]  GraphicShininess=75  DoExposeReferenceFrame=on  SerializedFrames=<Frames/>
  Plunger : sm_lib/Body Elements/Cylindrical Solid  CylinderRadius=plgB_rad  CylinderRadiusUnits=m  CylinderLength=plgB_len  CylinderLengthUnits=m  ExportEntireGeometry=off  InertiaType=CalculateFromGeometry  BasedOnType=Density  Density=plg_rho  DensityUnits=kg/m^3  Mass=1  MassUnits=kg  CenterOfMass=[0 0 0]  CenterOfMassUnits=m  MomentsOfInertia=[1 1 1]  MomentsOfInertiaUnits=kg*m^2  ProductsOfInertia=[1 1 1]  ProductsOfInertiaUnits=kg*m^2  GraphicType=FromGeometry  MarkerShape=Sphere  MarkerSize=10  GraphicVisPropType=SimpleVisualProperties  GraphicDiffuseColor=plg_clr  GraphicOpacity=plg_opc  GraphicSpecularColor=[0.5 0.5 0.5 1.0]  GraphicAmbientColor=[0.15 0.15 0.15 1.0]  GraphicEmissiveColor=[0.0 0.0 0.0 1.0]  GraphicShininess=75  DoExposeReferenceFrame=on  SerializedFrames=<Frames/>
  Seal Leak Visual : sm_lib/Body Elements/Cylindrical Solid  CylinderRadius=seal_leak_vis_rad  CylinderRadiusUnits=m  CylinderLength=seal_leak_vis_len  CylinderLengthUnits=m  ExportEntireGeometry=off  InertiaType=CalculateFromGeometry  BasedOnType=Density  Density=0.0001  DensityUnits=kg/m^3  Mass=1  MassUnits=kg  CenterOfMass=[0 0 0]  CenterOfMassUnits=m  MomentsOfInertia=[1 1 1]  MomentsOfInertiaUnits=kg*m^2  ProductsOfInertia=[1 1 1]  ProductsOfInertiaUnits=kg*m^2  GraphicType=FromGeometry  MarkerShape=Sphere  MarkerSize=10  GraphicVisPropType=SimpleVisualProperties  GraphicDiffuseColor=seal_leak_vis_clr  GraphicOpacity=seal_leak_vis_opc  GraphicSpecularColor=[0.5 0.5 0.5 1.0]  GraphicAmbientColor=[0.15 0.15 0.15 1.0]  GraphicEmissiveColor=[0.0 0.0 0.0 1.0]  GraphicShininess=75  DoExposeReferenceFrame=on  SerializedFrames=<Frames/>
  Stem : sm_lib/Body Elements/Cylindrical Solid  CylinderRadius=stem_rad  CylinderRadiusUnits=m  CylinderLength=stem_len  CylinderLengthUnits=m  ExportEntireGeometry=off  InertiaType=CalculateFromGeometry  BasedOnType=Density  Density=plg_rho  DensityUnits=kg/m^3  Mass=1  MassUnits=kg  CenterOfMass=[0 0 0]  CenterOfMassUnits=m  MomentsOfInertia=[1 1 1]  MomentsOfInertiaUnits=kg*m^2  ProductsOfInertia=[1 1 1]  ProductsOfInertiaUnits=kg*m^2  GraphicType=FromGeometry  MarkerShape=Sphere  MarkerSize=10  GraphicVisPropType=SimpleVisualProperties  GraphicDiffuseColor=plg_clr  GraphicOpacity=plg_opc  GraphicSpecularColor=[0.5 0.5 0.5 1.0]  GraphicAmbientColor=[0.15 0.15 0.15 1.0]  GraphicEmissiveColor=[0.0 0.0 0.0 1.0]  GraphicShininess=75  DoExposeReferenceFrame=on  SerializedFrames=<Frames/>
  Transform Cup Floor : sm_lib/Frames and Transforms/Rigid Transform  RotationMethod=None  FollAlignAxisA=+X  BaseAlignAxisA=+Y  FollAlignAxisB=+Y  BaseAlignAxisB=+Z  RotationStandardAxis=+Z  RotationAngle=0.0  RotationAngleUnits=deg  RotationArbitraryAxis=[0 0 1]  RotationSequenceAxes=FollowerAxes  RotationSequence=XYX  RotationSequenceAngles=[0 0 0]  RotationSequenceAnglesUnits=deg  RotationMatrix=[1 0 0; 0 1 0; 0 0 1]  Quaternion=[1 0 0 0]  TranslationMethod=StandardAxis  TranslationCartesianOffset=[0 0 0]  TranslationCartesianOffsetUnits=m  TranslationStandardAxis=+Z  TranslationStandardOffset=stem_len/2+cup_thk/2  TranslationStandardOffsetUnits=m  TranslationROffset=0  TranslationROffsetUnits=m  TranslationThetaOffset=0  TranslationThetaOffsetUnits=deg  TranslationZOffset=0  TranslationZOffsetUnits=m
  Transform Cup Wall : sm_lib/Frames and Transforms/Rigid Transform  RotationMethod=None  FollAlignAxisA=+X  BaseAlignAxisA=+Y  FollAlignAxisB=+Y  BaseAlignAxisB=+Z  RotationStandardAxis=+Z  RotationAngle=0.0  RotationAngleUnits=deg  RotationArbitraryAxis=[0 0 1]  RotationSequenceAxes=FollowerAxes  RotationSequence=XYX  RotationSequenceAngles=[0 0 0]  RotationSequenceAnglesUnits=deg  RotationMatrix=[1 0 0; 0 1 0; 0 0 1]  Quaternion=[1 0 0 0]  TranslationMethod=StandardAxis  TranslationCartesianOffset=[0 0 0]  TranslationCartesianOffsetUnits=m  TranslationStandardAxis=+Z  TranslationStandardOffset=stem_len/2+cup_len/2  TranslationStandardOffsetUnits=m  TranslationROffset=0  TranslationROffsetUnits=m  TranslationThetaOffset=0  TranslationThetaOffsetUnits=deg  TranslationZOffset=0  TranslationZOffsetUnits=m
  Transform Plunger Ctr : sm_lib/Frames and Transforms/Rigid Transform  RotationMethod=None  FollAlignAxisA=+X  BaseAlignAxisA=+Y  FollAlignAxisB=+Y  BaseAlignAxisB=+Z  RotationStandardAxis=+Z  RotationAngle=0.0  RotationAngleUnits=deg  RotationArbitraryAxis=[0 0 1]  RotationSequenceAxes=FollowerAxes  RotationSequence=XYX  RotationSequenceAngles=[0 0 0]  RotationSequenceAnglesUnits=deg  RotationMatrix=[1 0 0; 0 1 0; 0 0 1]  Quaternion=[1 0 0 0]  TranslationMethod=StandardAxis  TranslationCartesianOffset=[0 0 0]  TranslationCartesianOffsetUnits=m  TranslationStandardAxis=+Z  TranslationStandardOffset=plgB_len/2  TranslationStandardOffsetUnits=m  TranslationROffset=0  TranslationROffsetUnits=m  TranslationThetaOffset=0  TranslationThetaOffsetUnits=deg  TranslationZOffset=0  TranslationZOffsetUnits=m
  Transform Stem Ctr : sm_lib/Frames and Transforms/Rigid Transform  RotationMethod=None  FollAlignAxisA=+X  BaseAlignAxisA=+Y  FollAlignAxisB=+Y  BaseAlignAxisB=+Z  RotationStandardAxis=+Z  RotationAngle=0.0  RotationAngleUnits=deg  RotationArbitraryAxis=[0 0 1]  RotationSequenceAxes=FollowerAxes  RotationSequence=XYX  RotationSequenceAngles=[0 0 0]  RotationSequenceAnglesUnits=deg  RotationMatrix=[1 0 0; 0 1 0; 0 0 1]  Quaternion=[1 0 0 0]  TranslationMethod=StandardAxis  TranslationCartesianOffset=[0 0 0]  TranslationCartesianOffsetUnits=m  TranslationStandardAxis=+Z  TranslationStandardOffset=plgB_len/2+stem_len/2  TranslationStandardOffsetUnits=m  TranslationROffset=0  TranslationROffsetUnits=m  TranslationThetaOffset=0  TranslationThetaOffsetUnits=deg  TranslationZOffset=0  TranslationZOffsetUnits=m
  Transform Pin : sm_lib/Frames and Transforms/Rigid Transform  RotationMethod=StandardAxis  FollAlignAxisA=+X  BaseAlignAxisA=+Y  FollAlignAxisB=+Y  BaseAlignAxisB=+Z  RotationStandardAxis=+Y  RotationAngle=90  RotationAngleUnits=deg  RotationArbitraryAxis=[0 0 1]  RotationSequenceAxes=FollowerAxes  RotationSequence=XYX  RotationSequenceAngles=[0 0 0]  RotationSequenceAnglesUnits=deg  RotationMatrix=[1 0 0; 0 1 0; 0 0 1]  Quaternion=[1 0 0 0]  TranslationMethod=StandardAxis  TranslationCartesianOffset=[0 0 0]  TranslationCartesianOffsetUnits=m  TranslationStandardAxis=+Z  TranslationStandardOffset=stem_len/2+cup_pinOffset  TranslationStandardOffsetUnits=m  TranslationROffset=0  TranslationROffsetUnits=m  TranslationThetaOffset=0  TranslationThetaOffsetUnits=deg  TranslationZOffset=0  TranslationZOffsetUnits=m
  C : PMIOPort  Side=Left
  P : PMIOPort  Port=2  Side=Right
  connections:
  Transform Stem Ctr/RConn1 -- Transform Cup Wall/LConn1 -- Transform Pin/LConn1 -- Transform Cup Floor/LConn1 -- Stem/RConn1
  Transform Plunger Ctr/LConn1 -- C/RConn1
  Transform Plunger Ctr/RConn1 -- Seal Leak Visual/RConn1 -- Transform Stem Ctr/LConn1 -- Plunger/RConn1
  Cup Floor/RConn1 -- Transform Cup Floor/RConn1
  Cup Wall/RConn1 -- Transform Cup Wall/RConn1
  Transform Pin/RConn1 -- P/RConn1 -- Pin/RConn1

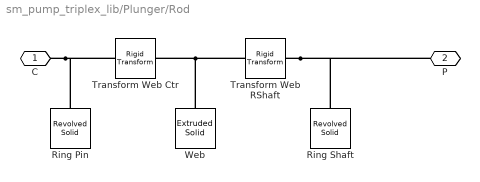
== system sm_pump_triplex_lib/Plunger/Rod ==
  Ring Pin : sm_lib/Body Elements/Revolved Solid  RevolutionCrossSection=conrod_ringP_xc_rev  RevolutionCrossSectionUnits=m  RevolutionExtent=Full  RevolutionAngle=180  RevolutionAngleUnits=deg  ExportConvexHullGeometry=off  InertiaType=CalculateFromGeometry  BasedOnType=Density  Density=conrod_rho  DensityUnits=kg/m^3  Mass=1  MassUnits=kg  CenterOfMass=[0 0 0]  CenterOfMassUnits=m  MomentsOfInertia=[1 1 1]  MomentsOfInertiaUnits=kg*m^2  ProductsOfInertia=[1 1 1]  ProductsOfInertiaUnits=kg*m^2  GraphicType=FromGeometry  MarkerShape=Sphere  MarkerSize=10  GraphicVisPropType=SimpleVisualProperties  GraphicDiffuseColor=conrod_clr  GraphicOpacity=conrod_opc  GraphicSpecularColor=[0.5 0.5 0.5 1.0]  GraphicAmbientColor=[0.15 0.15 0.15 1.0]  GraphicEmissiveColor=[0.0 0.0 0.0 1.0]  GraphicShininess=75  DoExposeReferenceFrame=on  SerializedFrames=<Frames/>
  Ring Shaft : sm_lib/Body Elements/Revolved Solid  RevolutionCrossSection=conrod_ringC_xc_rev  RevolutionCrossSectionUnits=m  RevolutionExtent=Full  RevolutionAngle=180  RevolutionAngleUnits=deg  ExportConvexHullGeometry=off  InertiaType=CalculateFromGeometry  BasedOnType=Density  Density=conrod_rho  DensityUnits=kg/m^3  Mass=1  MassUnits=kg  CenterOfMass=[0 0 0]  CenterOfMassUnits=m  MomentsOfInertia=[1 1 1]  MomentsOfInertiaUnits=kg*m^2  ProductsOfInertia=[1 1 1]  ProductsOfInertiaUnits=kg*m^2  GraphicType=FromGeometry  MarkerShape=Sphere  MarkerSize=10  GraphicVisPropType=SimpleVisualProperties  GraphicDiffuseColor=conrod_clr  GraphicOpacity=conrod_opc  GraphicSpecularColor=[0.5 0.5 0.5 1.0]  GraphicAmbientColor=[0.15 0.15 0.15 1.0]  GraphicEmissiveColor=[0.0 0.0 0.0 1.0]  GraphicShininess=75  DoExposeReferenceFrame=on  SerializedFrames=<Frames/>
  Transform Web Ctr : sm_lib/Frames and Transforms/Rigid Transform  RotationMethod=None  FollAlignAxisA=+X  BaseAlignAxisA=+Y  FollAlignAxisB=+Y  BaseAlignAxisB=+Z  RotationStandardAxis=+Z  RotationAngle=0.0  RotationAngleUnits=deg  RotationArbitraryAxis=[0 0 1]  RotationSequenceAxes=FollowerAxes  RotationSequence=XYX  RotationSequenceAngles=[0 0 0]  RotationSequenceAnglesUnits=deg  RotationMatrix=[1 0 0; 0 1 0; 0 0 1]  Quaternion=[1 0 0 0]  TranslationMethod=StandardAxis  TranslationCartesianOffset=[0 0 0]  TranslationCartesianOffsetUnits=m  TranslationStandardAxis=-X  TranslationStandardOffset=conrod_web_offP+conrod_web_len/2  TranslationStandardOffsetUnits=m  TranslationROffset=0  TranslationROffsetUnits=m  TranslationThetaOffset=0  TranslationThetaOffsetUnits=deg  TranslationZOffset=0  TranslationZOffsetUnits=m
  Transform Web RShaft : sm_lib/Frames and Transforms/Rigid Transform  RotationMethod=None  FollAlignAxisA=+X  BaseAlignAxisA=+Y  FollAlignAxisB=+Y  BaseAlignAxisB=+Z  RotationStandardAxis=+Z  RotationAngle=0.0  RotationAngleUnits=deg  RotationArbitraryAxis=[0 0 1]  RotationSequenceAxes=FollowerAxes  RotationSequence=XYX  RotationSequenceAngles=[0 0 0]  RotationSequenceAnglesUnits=deg  RotationMatrix=[1 0 0; 0 1 0; 0 0 1]  Quaternion=[1 0 0 0]  TranslationMethod=StandardAxis  TranslationCartesianOffset=[0 0 0]  TranslationCartesianOffsetUnits=m  TranslationStandardAxis=-X  TranslationStandardOffset=conrod_web_offC+conrod_web_len/2  TranslationStandardOffsetUnits=m  TranslationROffset=0  TranslationROffsetUnits=m  TranslationThetaOffset=0  TranslationThetaOffsetUnits=deg  TranslationZOffset=0  TranslationZOffsetUnits=m
  Web : sm_lib/Body Elements/Extruded Solid  ExtrusionType=General  PolygonNumSides=3  PolygonOuterRadius=1  PolygonOuterRadiusUnits=m  ExportEntireGeometry=off  ExtrusionCrossSection=conrod_web_xc  ExtrusionCrossSectionUnits=m  ExportConvexHullGeometry=off  ExtrusionLength=conrod_thk  ExtrusionLengthUnits=m  InertiaType=CalculateFromGeometry  BasedOnType=Density  Density=conrod_rho  DensityUnits=kg/m^3  Mass=1  MassUnits=kg  CenterOfMass=[0 0 0]  CenterOfMassUnits=m  MomentsOfInertia=[1 1 1]  MomentsOfInertiaUnits=kg*m^2  ProductsOfInertia=[1 1 1]  ProductsOfInertiaUnits=kg*m^2  GraphicType=FromGeometry  MarkerShape=Sphere  MarkerSize=10  GraphicVisPropType=SimpleVisualProperties  GraphicDiffuseColor=conrod_clr  GraphicOpacity=conrod_opc  GraphicSpecularColor=[0.5 0.5 0.5 1.0]  GraphicAmbientColor=[0.15 0.15 0.15 1.0]  GraphicEmissiveColor=[0.0 0.0 0.0 1.0]  GraphicShininess=75  DoExposeReferenceFrame=on  SerializedFrames=<Frames/>
  C : PMIOPort  Side=Left
  P : PMIOPort  Port=2  Side=Right
  connections:
  Transform Web RShaft/RConn1 -- P/RConn1 -- Ring Shaft/RConn1
  Web/RConn1 -- Transform Web RShaft/LConn1 -- Transform Web Ctr/RConn1
  C/RConn1 -- Ring Pin/RConn1 -- Transform Web Ctr/LConn1

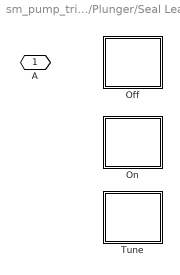
== system sm_pump_triplex_lib/Plunger/Seal Leak ==
  Off : Subsystem  VariantControl=Off
      mask Display: image('sm_pump_triplex_Seal_Leak_Off_IMAGE.png');
  On : Subsystem  VariantControl=On
      mask Display: image('sm_pump_triplex_Seal_Leak_On_IMAGE.png');
  Tune : Subsystem  VariantControl=Tune
      mask Display: image('sm_pump_triplex_Seal_Leak_On_IMAGE.png');
  " A " : PMIOPort  Side=Left

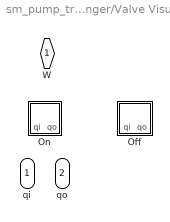
== system sm_pump_triplex_lib/Plunger/Valve Visual ==
  "qi " : Inport
  "qo " : Inport  Port=2
  Off : Subsystem  VariantControl=Off
      mask Display: disp(' ');
  On : Subsystem  VariantControl=On
      mask Display: image('sm_pump_triplex_Valve_Vis_IMAGE.png');
  " W " : PMIOPort  Side=Right

== system sm_pump_triplex_lib/Plunger/Seal Leak/Off ==
  A : PMIOPort  Side=Left
